simulink model "non_ACC"  (R2021b)
settings: Solver=ode5  StartTime=0.0  StopTime=90  FixedStep=1/20  RelTol=1e-3
PreLoadFcn:
  | mbxruntime.callbacks.PreLoadFcn(bdroot);
PostLoadFcn:
  | mbxruntime.callbacks.PostLoadFcn(bdroot);
InitFcn:
  | mbxruntime.callbacks.InitFcn(bdroot);
StartFcn:
  | mbxruntime.callbacks.StartFcn(bdroot);
StopFcn:
  | mbxruntime.callbacks.StopFcn(bdroot);
model workspace: external: MAT-File .\kea_demo_0218_cs_hws.mat (data not in the file)
undefined symbols (not defined in the file): DiscIntNeverNeededParam, kea_demo_0218_cs_1d5c9b61e8e009e5, kea_demo_0218_cs_4669f259e7287783, kea_demo_0218_cs_87ee11d7829c0052, kea_demo_0218_cs_Audi_A3_1_Dynamics_Simple_initialPitch, kea_demo_0218_cs_Audi_A3_1_Dynamics_Simple_initialRoll, kea_demo_0218_cs_Audi_A3_1_Dynamics_Simple_initialX, kea_demo_0218_cs_Audi_A3_1_Dynamics_Simple_initialY, kea_demo_0218_cs_Audi_A3_1_Dynamics_Simple_initialYaw, kea_demo_0218_cs_Audi_A3_1_Dynamics_Simple_initialZ, kea_demo_0218_cs_Audi_A3_1_PathFollower_Preview_1_PathUniqueID, kea_demo_0218_cs_Roewe_550_S_Sedan_1_Dynamics_Simple_initialX, kea_demo_0218_cs_Roewe_550_S_Sedan_1_Dynamics_Simple_initialY, kea_demo_0218_cs_Roewe_550_S_Sedan_1_Dynamics_Simple_initialYaw, kea_demo_0218_cs_Roewe_550_S_Sedan_1_Dynamics_Simple_initialZ, mbxruntime, warningInitialVelocity, x0
libraries: simulink x56, simulink_extras x18
(part 1 of 7)
CloseFcn:
  | mbxruntime.callbacks.CloseFcn(bdroot);
settings Model: PacingRate=10  Creator=PRESCAN  LastModifiedBy=PRO
settings SolverCC: AlgebraicLoopSolver=TrustRegion
settings DataIOCC: LimitDataPoints=on  SaveFormat=Array  SignalLoggingSaveFormat=ModelDataLogs  ReturnWorkspaceOutputs=off
settings OptimizationCC: DefaultParameterBehavior=Inlined  ExpressionDepthLimit=2147483647  InitFltsAndDblsToZero=on  LifeSpan=inf
settings DebuggingCC: SaveWithParameterizedLinksMsg=none  UnderspecifiedInitializationDetection=Classic  MergeDetectMultiDrivingBlocksExec=none  SignalResolutionControl=TryResolveAllWithWarning  MultiTaskDSMMsg=warning  MultiTaskCondExecSysMsg=none  FcnCallInpInsideContextMsg=warning  AllowSymbolicDim=off  StateNameClashWarn=warning  SFUnexpectedBacktrackingDiag=warning  SFNoUnconditionalDefaultTransitionDiag=warning  SFExecutionAtInitializationDiag=none  SFMachineParentedDataDiag=warning  ArithmeticOperatorsInVariantConditions=warning
settings HardwareCC: ProdBitPerPointer=32  ProdBitPerSizeT=32  ProdBitPerPtrDiffT=32  ProdLargestAtomicFloat=None  ProdIntDivRoundTo=Undefined  ProdEndianess=Unspecified  ProdWordSize=32  ProdHWDeviceType=32-bit Generic
settings ModelReferenceCC: UpdateModelReferenceTargets=IfOutOfDate  PropagateSignalLabelsOutOfModel=off
settings SFSimCC: SimUseLocalCustomCode=off  SimParseCustomCode=off  CustomCodeUndefinedFunction=UseInterfaceOnly
settings SFSimCC: SimCustomHeaderCode=|
  | #include "prescan.h"
  | #include "prescan_platform.h"
settings RTWCC: RTWUseLocalCustomCode=off
settings CodeAppCC: StateflowObjectComments=on
settings GRTTargetCC: TargetFcnLib=ansi_tfl_tmw.mat  TargetLangStandard=C89/C90 (ANSI)  CombineOutputUpdateFcns=off  GRTInterface=on
settings ConfigComp: CovMetricSettings=dw  CovSaveCumulativeToWorkspaceVar=on  CovSaveSingleToWorkspaceVar=on  CovExternalEMLEnable=off  CovSFcnEnable=off

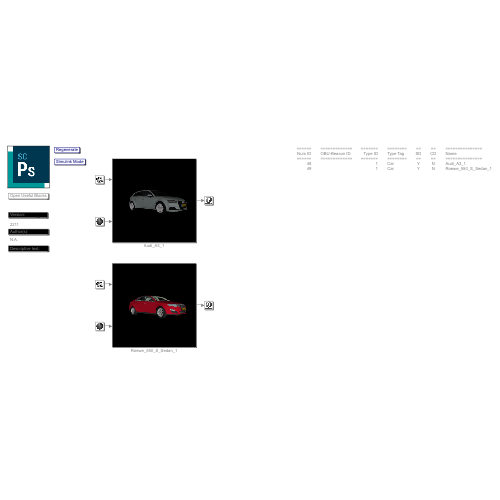
[thumbnail: Simulink's stored preview of the top-level diagram]
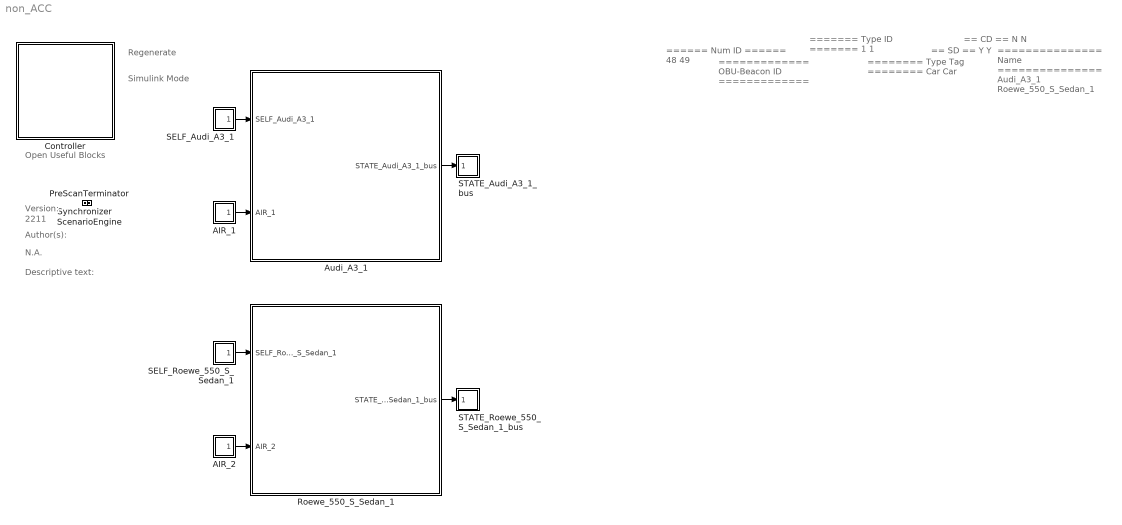
== system non_ACC ==
  note: Regenerate
  note: Simulink Mode
  note: Open Useful Blocks
  note: 2211
  note: Version:
  note: Author(s):
  note: N.A.
  note: Descriptive text:
  note: ======
      | Num ID
      | ======
      | 48
      | 49
  note: =============
      | OBU-Beacon ID
      | =============
  note: =======
      | Type ID
      | =======
      | 1
      | 1
  note: ========
      | Type Tag
      | ========
      | Car
      | Car
  note: ==
      | SD
      | ==
      | Y
      | Y
  note: ==
      | CD
      | ==
      | N
      | N
  note: ===============
      | Name
      | ===============
      | Audi_A3_1
      | Roewe_550_S_Sedan_1
  AIR_1 : Subsystem  Tag=sensor/AIR  Priority=30  LoadFcn=load('PrescanAIRSensorData.mat');load('PrescanAIRSensorMessage.mat')  mask(PreScan Source Block: Actor Independent Receiver (AIR)){}
      mask help:
      | The Actor Information Receiver sensor provides a fast, simple and generic detection solution which is not tied up to a specific technology. The AIR detects the intersection point of the bounding box with the straight line from the sensor axis system to the middle of the bounding box.
      |
      | For more information, please click Help.
      settings: OpenFcn=open_system([gcb '/Sensor'],'mask')
      mask Help: eval('openHelp(413)')
      mask Display: image(imread('AIR.png'))
  AIR_2 : Subsystem  Tag=sensor/AIR  Priority=30  LoadFcn=load('PrescanAIRSensorData.mat');load('PrescanAIRSensorMessage.mat')  mask(PreScan Source Block: Actor Independent Receiver (AIR)){}
      mask help:
      | The Actor Information Receiver sensor provides a fast, simple and generic detection solution which is not tied up to a specific technology. The AIR detects the intersection point of the bounding box with the straight line from the sensor axis system to the middle of the bounding box.
      |
      | For more information, please click Help.
      settings: OpenFcn=open_system([gcb '/Sensor'],'mask')
      mask Help: eval('openHelp(413)')
      mask Display: image(imread('AIR.png'))
  Audi_A3_1 : Subsystem  Tag=WorldObjectSubSystem  InitFcn=UniqueId = '189';
      mask init:
      | modelPath = GenericModelHelper.getGenericModelFilePath('ModelDepo','Vehicles\Audi_A3\Audi_A3.pgmb','904257d8a4712c49871b2bb1a5c4c7b1');imagePath = GenericModelHelper.getCompilationPicture(modelPath, 'Audi_A3.png');
      mask Display: image(imread(imagePath));color('white');text(0, 0, ' ID=48\n')
  Controller : Subsystem  Description=8A3CD2955739A82C886C20AE3E253D78460D53180EE2C1B14CC08DF75A70BE77  Priority=-1  LoadFcn=load PreScanControllerData  mask(PreScan Simulation Controller){prescanversion='2022.3.0', ModelReferencing=off, TimeStep=1/20, ControlMode=0, PreScanExecutionMode=on, ControllerCount=0, ControllerIndex=0, ControllerOptions=''}
      mask prompts: prescanversion "Prescan Version"; ModelReferencing "Use Model Referencing"; TimeStep "Upload Period [s]"; ControlMode "Control Mode"; PreScanExecutionMode "Execution Mode"; ControllerCount "Controller Count"; ControllerIndex "Controller Index"; ControllerOptions "Controller Options"
      mask help:
      | Please do not remove this block from the compilation sheet,
      | as it connects the model to the Prescan environment.
      mask init:
      | model = bdroot(gcb);
      | ExperimentFile = mbxruntime.findExperimentFile(model,true); %relative path
      | 
      | [d1, d2, prescandata] = prescan_Settings();
      | ModelDepo = fullfile(prescandata,'ModelDepo'); 
      | 
      | RTmode = mbxruntime.getRTMode(model);
      | 
      | SimulationMode = get_param(bdroot,'SimulationMode');
      | if strcmp(SimulationMode, 'rapid-accelerator')
      |     SimulationMode = 'external';
      | end
      | TargetName = get_param(bdroot,'SystemTargetFile');
      settings: ModelCloseFcn=assignin('base',['model_closed_' bdroot],true);
      mask Help: eval('openHelp(812)')
      mask Display: image(imread('prescanlogo.ico'))
  PreScanTerminator : Subsystem  Tag=PreScanTerminator  Priority=999  LoadFcn=load PrescanTerminatorData  mask(PreScan Simulation Terminator){TimeStep=1/20}
      mask prompts: TimeStep "Upload Period [s]"
      mask help:
      | Please do not remove this block from the compilation sheet as it
      | connects the model to the PreScan environment.
      mask Help: eval('openHelp(812)')
      mask Display: image(imread('prescanlogo.ico'))
  Roewe_550_S_Sedan_1 : Subsystem  Tag=WorldObjectSubSystem  InitFcn=UniqueId = '192';
      mask init:
      | modelPath = GenericModelHelper.getGenericModelFilePath('ModelDepo','Vehicles\Roewe_550_S\Roewe_550_S.pgmb','e36b3c1cdc77adba028a993f0879aa02');imagePath = GenericModelHelper.getCompilationPicture(modelPath, 'Roewe_550_S_HighPoly.png');
      mask Display: image(imread(imagePath));color('white');text(0, 0, ' ID=49\n')
  SELF_Audi_A3_1 : Subsystem  Tag=sensor/SelfPort  Priority=30  LoadFcn=load('PreScanSelfSensorData.mat')  mask(PreScan Source Block: SELF){}
      mask help:
      | The SELF port shows (state) information of the actor itself. The outputs are position in the experiment's axis system and the GPS coordinates, and the object's absolute velocity and compass heading.
      |
      | For more information, please click Help.
      settings: OpenFcn=open_system([gcb '/Sensor'],'mask')
      mask Help: eval('openHelp(462)')
      mask Display: image(imread('GPS.png'))
  SELF_Roewe_550_S_Sedan_1 : Subsystem  Tag=sensor/SelfPort  Priority=30  LoadFcn=load('PreScanSelfSensorData.mat')  mask(PreScan Source Block: SELF){}
      mask help:
      | The SELF port shows (state) information of the actor itself. The outputs are position in the experiment's axis system and the GPS coordinates, and the object's absolute velocity and compass heading.
      |
      | For more information, please click Help.
      settings: OpenFcn=open_system([gcb '/Sensor'],'mask')
      mask Help: eval('openHelp(462)')
      mask Display: image(imread('GPS.png'))
  STATE_Audi_A3_1_bus : Subsystem  Tag=actuator/StatePort  Priority=0  LoadFcn=load('PreScanStateActuatorData.mat')  mask(PreScan Sink Block: State){}
      mask help:
      | The Actor State contains a vector signal of size (9x1), containing the following signals:
      |
      | -  Position    	(x,y,z)             	[m]
      | -  Velocity    	(vx,vy,vz)         	[m/s]
      | -  Angles       	(Roll, Pitch, Yaw)	[rad]
      |
      | The Actor state is defined in the global axis system.
      | The state is superponed on the Initial position defined in the GUI.
      |
      | For more information, please click Help.
      settings: OpenFcn=open_system([gcb '/Actuator'],'mask')
      mask Help: eval('openHelp(222)')
      mask Display: image(imread('State.png'))
  STATE_Roewe_550_S_Sedan_1_bus : Subsystem  Tag=actuator/StatePort  Priority=0  LoadFcn=load('PreScanStateActuatorData.mat')  mask(PreScan Sink Block: State){}
      mask help:
      | The Actor State contains a vector signal of size (9x1), containing the following signals:
      |
      | -  Position    	(x,y,z)             	[m]
      | -  Velocity    	(vx,vy,vz)         	[m/s]
      | -  Angles       	(Roll, Pitch, Yaw)	[rad]
      |
      | The Actor state is defined in the global axis system.
      | The state is superponed on the Initial position defined in the GUI.
      |
      | For more information, please click Help.
      settings: OpenFcn=open_system([gcb '/Actuator'],'mask')
      mask Help: eval('openHelp(222)')
      mask Display: image(imread('State.png'))
  ScenarioEngine : Subsystem  Tag=PreScanOpenScenarioBlock  Priority=10  LoadFcn=load PrescanSynchronizeData  mask(PreScan Simulation Core Block){TimeStep=1/20}
      mask prompts: TimeStep "Timestep [s]"
      mask help:
      | Please do not remove this block from the PreScan compilation sheet,
      | as it contains essential configuration parameters for a PreScan simulation.
      settings: DeleteFcn=PreScanBlockDeleteFcn;
      mask Display: image(imread('prescanlogo.ico'))
  Synchronizer : Subsystem  Tag=PreScanSynchronizer  Priority=20  LoadFcn=load PrescanSynchronizeData  mask(PreScan Simulation Core Block){TimeStep=1/20}
      mask prompts: TimeStep "Timestep [s]"
      mask help:
      | Please do not remove this block from the PreScan compilation sheet,
      | as it contains essential configuration parameters for a PreScan simulation.
      settings: DeleteFcn=PreScanBlockDeleteFcn;
      mask Display: image(imread('prescanlogo.ico'))
  wires:
  Audi_A3_1/1(STATE_Audi_A3_1_bus) -> STATE_Audi_A3_1_bus/1(STATE_Audi_A3_1_bus)
  SELF_Audi_A3_1/1(SELF_Audi_A3_1) -> Audi_A3_1/1(SELF_Audi_A3_1)
  AIR_1/1(AIR_1) -> Audi_A3_1/2(AIR_1)
  Roewe_550_S_Sedan_1/1(STATE_Roewe_550_S_Sedan_1_bus) -> STATE_Roewe_550_S_Sedan_1_bus/1(STATE_Roewe_550_S_Sedan_1_bus)
  SELF_Roewe_550_S_Sedan_1/1(SELF_Roewe_550_S_Sedan_1) -> Roewe_550_S_Sedan_1/1(SELF_Roewe_550_S_Sedan_1)
  AIR_2/1(AIR_2) -> Roewe_550_S_Sedan_1/2(AIR_2)

== system non_ACC/AIR_1 ==
  Sensor : S-Function  FunctionName=sfun_AIRSensor  Parameters=mbxruntime.parameters.convert(detectableObjects), mbxruntime.parameters.convert(sensorID), mbxruntime.parameters.convert(timestep)  SFunctionDeploymentMode=off  EnableBusSupport=off  mask(PreScan Source Block: Actor Independent Receiver (AIR)){detectableObjects=1, sensorID=190, timestep=1/20}
      mask prompts: detectableObjects "Max detectable objects"; sensorID "Sensor ID"; timestep "MATLAB timestep:"
      mask help:
      | The Actor Information Receiver sensor provides a fast, simple and generic detection solution which is not tied up to a specific technology. The AIR detects the intersection point of the bounding box with the straight line from the sensor axis system to the middle of the bounding box.
      |
      | For more information, please click Help.
      mask Help: eval('openHelp(413)')
      mask Display: image(imread('AIR.png'))
  AIR_1 : Outport  Tag=outport/AIR  OutDataTypeStr=Bus: PRESCAN_AIRSENSORMESSAGE  PortDimensions=1  SampleTime=1/20
  wires:
  Sensor/1 -> AIR_1/1

== system non_ACC/AIR_2 ==
  Sensor : S-Function  FunctionName=sfun_AIRSensor  Parameters=mbxruntime.parameters.convert(detectableObjects), mbxruntime.parameters.convert(sensorID), mbxruntime.parameters.convert(timestep)  SFunctionDeploymentMode=off  EnableBusSupport=off  mask(PreScan Source Block: Actor Independent Receiver (AIR)){detectableObjects=1, sensorID=193, timestep=1/20}
      mask prompts: detectableObjects "Max detectable objects"; sensorID "Sensor ID"; timestep "MATLAB timestep:"
      mask help:
      | The Actor Information Receiver sensor provides a fast, simple and generic detection solution which is not tied up to a specific technology. The AIR detects the intersection point of the bounding box with the straight line from the sensor axis system to the middle of the bounding box.
      |
      | For more information, please click Help.
      mask Help: eval('openHelp(413)')
      mask Display: image(imread('AIR.png'))
  AIR_2 : Outport  Tag=outport/AIR  OutDataTypeStr=Bus: PRESCAN_AIRSENSORMESSAGE  PortDimensions=1  SampleTime=1/20
  wires:
  Sensor/1 -> AIR_2/1

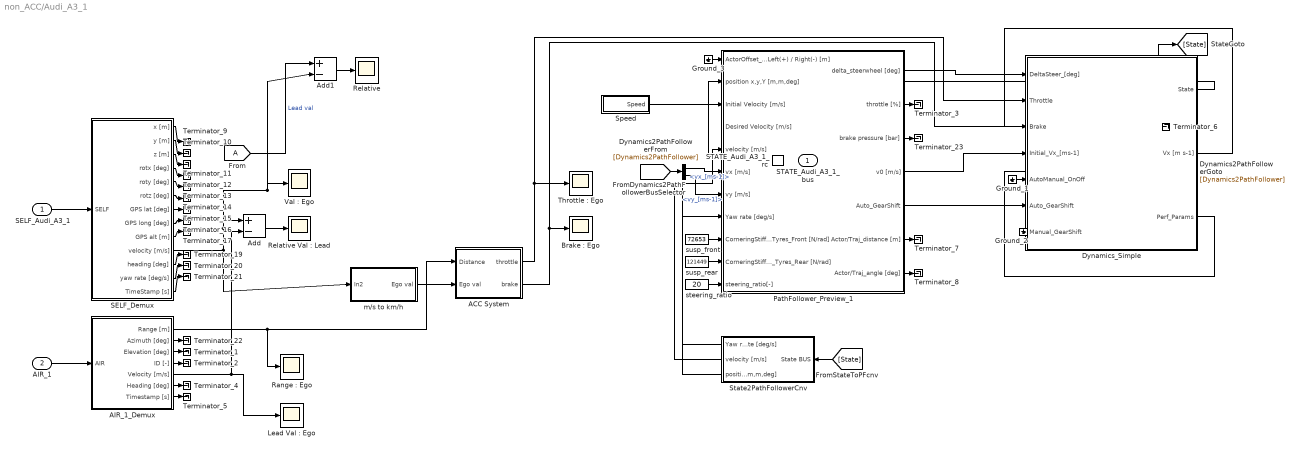
== system non_ACC/Audi_A3_1 ==
  SELF_Audi_A3_1 : Inport  Tag=inport/SelfPort  OutDataTypeStr=Bus: PRESCAN_SELFSENSORDATA  PortDimensions=1  SampleTime=1/20  BusOutputAsStruct=on
  AIR_1 : Inport  Tag=inport/AIR  Port=2  OutDataTypeStr=Bus: PRESCAN_AIRSENSORMESSAGE  PortDimensions=1  SampleTime=1/20  BusOutputAsStruct=on
  ACC System : Subsystem
  AIR_1_Demux : Subsystem  Tag=demux/AIR  mask(PreScan Demux Block: AIR){DetectionType=BBox, detectableObjects=1}
      mask prompts: DetectionType "Detection Type"; detectableObjects "Max. detectable objects"
      mask help:
      | The Actor Information Receiver sensor provides a fast, simple and generic detection solution which is not tied up to a specific technology and can be used for scenarios in which a simple sensor is needed.
      |
      | For more information, please click Help.
      mask init:
      | switch DetectionType
      |     case 1
      |         DetectionTypeStr = 'Center';
      |     case 2
      |         DetectionTypeStr = 'BBox';
      |     case 3
      |         DetectionTypeStr = 'CoG';
      |     otherwise
      |         DetectionTypeStr = 'Unknown';
      | end
      settings: DeleteFcn=PreScanBlockDeleteFcn;
      mask Help: eval('openHelp(413)')
      mask TypeOptions DetectionType: Center | BBox | CoG
      mask Display:
      | disp(char('Det. type:         ',['{\it',DetectionTypeStr,'}']),'texmode','on')
      | port_label('output',1,'Range [m]')
      | port_label('output',2,'{\theta} [deg]','texmode','on')
      | port_label('output',3,'{\phi} [deg]','texmode','on')
      | port_label('output',4,'ID [-]','texmode','on')
      | port_label('output',5,'Velocity [m/s]','texmode','on')
      | port_label('output',6,'Heading [deg]','texmode','on')
      | port_label('output',7,'Timestamp [s]','texmode','on')
  Add : Sum  Inputs=+-
  Add1 : Sum  Inputs=+-
  "Brake : Ego" : Scope
  Dynamics_Simple : Subsystem  Tag=Simple_Vehicle_Dynamics  mask(PreScan Block: Simple Dynamics){TimeStep=1/20, initialX=kea_demo_0218_cs_Audi_A3_1_Dynamics_Simple_initialX, initialY=kea_demo_0218_cs_Audi_A3_1_Dynamics_Simple_initialY, initialZ=kea_demo_0218_cs_Audi_A3_1_Dynamics_Simple_initialZ, initialRoll=kea_demo_0218_cs_Audi_A3_1_Dynamics_Simple_initialRoll, initialPitch=kea_demo_0218_cs_Audi_A3_1_Dynamics_Simple_initialPitch, initialYaw=kea_demo_0218_cs_Audi_A3_1_Dynamics_Simple_initialYaw}
      mask prompts: TimeStep "Auto assigned: Time Step [s]"; initialX "Ini x-position VEHICLE wrt GLOBAL axis system [m]"; initialY "Ini y-position VEHICLE wrt GLOBAL axis system [m]"; initialZ "Ini z-position VEHICLE wrt GLOBAL axis system [m]"; initialRoll "Ini roll-angle BODY wrt VEHICLE axis system [deg]"; initialPitch "Ini pitch-angle BODY wrt VEHICLE axis system [deg]"; initialYaw "Ini yaw-angle VEHICLE wrt GLOBAL axis system [deg]"
      mask help:
      | The Simple Dynamics Model is selected in the GUI to simulate vehicle dynamics behavior.
      |
      | The Simple Dynamics Model is completely open to the user. The parameters of this model can be set in the Simple Dynamics dialog in the GUI.
      |
      | For more information, please click Help.
      mask init:
      | p = SimpleDyn_pars;
      settings: DeleteFcn=PreScanBlockDeleteFcn;
      mask Help: eval('openHelp(220)')
      mask Display:
      | image(imread('SimpleDyn.png'))
      | port_label('input', 1, '{\delta}_S_t_ _e_e_r [deg]','texmode','on')
      | port_label('input', 2, 'Throttle [%]')
      | port_label('input', 3, 'Brake Pres [bar]')
      | port_label('input', 4, 'V_0 [ms-1]','texmode','on')
      | port_label('input', 5, 'Auto=[0]/Manual=[1]')
      | port_label('input', 6, 'Auto_GearShift')
      | port_label('input', 7, 'Manual_GearShift')
      | port_label('output', 1, 'State')
      | port_label('output', 2, 'Vx [ms-1]')
      | port_label('output', 3, 'Perf Params')
  FromDynamics2PathFollowerBusSelector : BusSelector  OutputSignals=vx_[ms-1],vy_[ms-1]
  Ground_1 : Ground
  Ground_2 : Ground
  Ground_3 : Ground
  "Lead Val : Ego" : Scope
  PathFollower_Preview_1 : Subsystem  Tag=PathFollower_Preview  LoadFcn=load PrescanXYZData;  mask(PreScan Block: Path Follower with Preview){LongCtrl_P=20, LongCtrl_I=0.3, LongCtrl_D=3.065, LongCtrl_AWU=1, LongCtrlDefault_P=20, LongCtrlDefault_I=0.3, LongCtrlDefault_D=3.065, LongCtrlDefault_AWU=1, PathUniqueID=kea_demo_0218_cs_Audi_A3_1_PathFollower_Preview_1_PathUniqueID, mass=1820, Jzz=3746, length_a=1.34, length_l=2.609, Angle_Max_SteeringWheel=500, PreviewTime=1, DelayTime=0.1, LowSpeedLimit=20, MaxSteeringRate=1200, CSSampleTime=1/20, PFIntegrationFrequency=20}
      mask prompts: LongCtrl_P "Longitudinal Controller P"; LongCtrl_I "Longitudinal Controller I"; LongCtrl_D "Longitudinal Controller D"; LongCtrl_AWU "Longitudinal Controller AWU"; PathUniqueID "Path Unique ID"; mass "Mass vehicle total [kg]"; Jzz "Inertia vehicle around yaw axis [kg m2]"; length_a "Distance between COG and front axle [m]"; length_l "Length of wheelbase [m]"; Angle_Max_SteeringWheel "Maximum steering wheel angle [deg]"; PreviewTime "Preview time [s]"; DelayTime "Delay time [s]"; LowSpeedLimit "Low-speed limit [km/h]"; MaxSteeringRate "Maximum steering wheel angle rate [deg/s]"; CSSampleTime "Compilation Sheet sample time [s]"; PFIntegrationFrequency "Lateral controller frequency [Hz]"
      mask help:
      | The Path Follower Model is selected in the GUI to simulate driver behavior.
      |
      | For more information, please click Help.
      mask init:
      | RefreshCounter = max(floor((1/CSSampleTime) / (PFIntegrationFrequency)), 1);
      | PathFollowerBlockPath = gcb;
      mask Help: eval('openHelp(233)')
      mask DialogControl Container12 Prompt: Controller Parameters
      mask DialogControl Control2 Prompt: Reset PID parameters
      mask DialogControl Control2 Callback:
      | LongCtrlDefault_P = get_param(gcb,'LongCtrlDefault_P');
      | set_param(gcb,'LongCtrl_P',LongCtrlDefault_P);
      | 
      | LongCtrlDefault_I = get_param(gcb,'LongCtrlDefault_I');
      | set_param(gcb,'LongCtrl_I',LongCtrlDefault_I);
      | 
      | LongCtrlDefault_D = get_param(gcb,'LongCtrlDefault_D');
      | set_param(gcb,'LongCtrl_D',LongCtrlDefault_D);
      | 
      | LongCtrlDefault_AWU = get_param(gcb,'LongCtrlDefault_AWU');
      | set_param(gcb,'LongCtrl_AWU',LongCtrlDefault_AWU);
      mask DialogControl Container10 Prompt: System Parameters
  "Range : Ego" : Scope
  Relative : Scope
  "Relative Val : Lead" : Scope
  SELF_Demux : Subsystem  Tag=demux/SelfPort  mask(PreScan Demux Block:){}
      mask help:
      | The SELF port shows (state) information of the actor itself. The outputs are position in the experiment's axis system and the GPS coordinates, and the object's absolute velocity and compass heading.
      |
      | For more information, please click Help.
      settings: DeleteFcn=PreScanBlockDeleteFcn;
      mask Help: eval('openHelp(462)')
      mask Display:
      | port_label('output',1,'x [m]')
      | port_label('output',2,'y [m]')
      | port_label('output',3,'z [m]','texmode','on')
      | port_label('output',4,'Rotx [deg]','texmode','on')
      | port_label('output',5,'Roty [deg]','texmode','on')
      | port_label('output',6,'Rotz [deg]','texmode','on')
      | port_label('output',7,'GPS lat [deg]','texmode','on')
      | port_label('output',8,'GPS long [deg]','texmode','on')
      | port_label('output',9,'GPS alt [m]','texmode','on')
      | port_label('output',10,'Velocity [m/s]')
      | port_label('output',11,'Heading [deg]')
      | port_label('output',12,'Yaw rate [deg/s]')
      | port_label('output',13,'Timestamp [s]')
  STATE_Audi_A3_1_rc : RateTransition  Tag=mux_rc/StatePort  OutPortSampleTimeOpt=Inherit
  Speed : Subsystem
      settings: OpenFcn=open_system([gcb '/sfun'],'mask')
  State2PathFollowerCnv : Subsystem  Tag=State2PFConnection/cnv
  Terminator_{1..17,19..23} (22 alike) : Terminator
  "Throttle : Ego" : Scope
  "Val : Ego" : Scope
  m/s to km/h : Subsystem
  steering_ratio : Constant  Tag=steering_ratio  Value=20
  susp_front : Constant  Tag=susp_front  Value=72653
  susp_rear : Constant  Tag=susp_rear  Value=121449
  STATE_Audi_A3_1_bus : Outport  Tag=outport/StatePort  OutDataTypeStr=Bus: PRESCAN_STATEACTUATORDATA  PortDimensions=1  SampleTime=1/20
  wires:
  STATE_Audi_A3_1_rc/1 -> STATE_Audi_A3_1_bus/1
  SELF_Audi_A3_1/1 -> SELF_Demux/1(SELF)
  AIR_1/1 -> AIR_1_Demux/1(AIR)
  susp_front/1 -> PathFollower_Preview_1/9(CorneringStiffness_Tyres_Front [N/rad])
  susp_rear/1 -> PathFollower_Preview_1/10(CorneringStiffness_Tyres_Rear [N/rad])
  steering_ratio/1 -> PathFollower_Preview_1/11(steering_ratio[-])
  Speed/1(Speed) -> PathFollower_Preview_1/3(Initial Velocity [m/s])
  Dynamics_Simple/1(State) -> STATE_Audi_A3_1_rc/1, [State]
  [State] -> State2PathFollowerCnv/1(State BUS)
  State2PathFollowerCnv/1(Yaw rate [deg/s]) -> PathFollower_Preview_1/8(Yaw rate [deg/s])
  State2PathFollowerCnv/2(velocity [m/s]) -> PathFollower_Preview_1/5(velocity [m/s])
  State2PathFollowerCnv/3(position x,y,Y [m,m,deg]) -> PathFollower_Preview_1/2(position x,y,Y [m,m,deg])
  PathFollower_Preview_1/1(delta_steerwheel [deg]) -> Dynamics_Simple/1(DeltaSteer_[deg])
  PathFollower_Preview_1/2(throttle [%]) -> Terminator_3/1
  PathFollower_Preview_1/3(brake pressure [bar]) -> Terminator_23/1
  PathFollower_Preview_1/4(v0 [m/s]) -> Dynamics_Simple/4(Initial_Vx_[ms-1])
  PathFollower_Preview_1/5(Auto_GearShift) -> Dynamics_Simple/6(Auto_GearShift)
  Dynamics_Simple/3(Perf_Params) -> [Dynamics2PathFollower]
  FromDynamics2PathFollowerBusSelector/1 -> PathFollower_Preview_1/6(vx [m/s])  "<vx_[ms-1]>"
  FromDynamics2PathFollowerBusSelector/2 -> PathFollower_Preview_1/7(vy [m/s])  "<vy_[ms-1]>"
  [Dynamics2PathFollower] -> FromDynamics2PathFollowerBusSelector/1
  AIR_1_Demux/3(Elevation [deg]) -> Terminator_1/1
  AIR_1_Demux/4(ID [-]) -> Terminator_2/1
  AIR_1_Demux/6(Heading [deg]) -> Terminator_4/1
  AIR_1_Demux/7(Timestamp [s]) -> Terminator_5/1
  Ground_1/1 -> Dynamics_Simple/5(AutoManual_OnOff)
  Ground_2/1 -> Dynamics_Simple/7(Manual_GearShift)
  Dynamics_Simple/2(Vx [m s-1]) -> Terminator_6/1
  Ground_3/1 -> PathFollower_Preview_1/1(ActorOffset_Left(+) / Right(-) [m])
  PathFollower_Preview_1/6(Actor/Traj_distance [m]) -> Terminator_7/1
  PathFollower_Preview_1/7(Actor/Traj_angle [deg]) -> Terminator_8/1
  SELF_Demux/1(x [m]) -> Terminator_9/1
  SELF_Demux/2(y [m]) -> Terminator_10/1
  SELF_Demux/3(z [m]) -> Terminator_11/1
  SELF_Demux/4(rotx [deg]) -> Terminator_12/1
  SELF_Demux/5(roty [deg]) -> Terminator_13/1
  SELF_Demux/6(rotz [deg]) -> Terminator_14/1
  SELF_Demux/7(GPS lat [deg]) -> Terminator_15/1
  SELF_Demux/8(GPS long [deg]) -> Terminator_16/1
  SELF_Demux/9(GPS alt [m]) -> Terminator_17/1
  SELF_Demux/11(heading [deg]) -> Terminator_19/1
  SELF_Demux/12(yaw rate [deg/s]) -> Terminator_20/1
  SELF_Demux/13(TimeStamp [s]) -> Terminator_21/1
  AIR_1_Demux/2(Azimuth [deg]) -> Terminator_22/1
  AIR_1_Demux/1(Range [m]) -> "Range : Ego"/1, ACC System/1(Distance)
  ACC System/1(throttle) -> Dynamics_Simple/2(Throttle), "Throttle : Ego"/1
  ACC System/2(brake) -> Dynamics_Simple/3(Brake), "Brake : Ego"/1
  m/s to km/h/1(Ego val) -> ACC System/2(Ego val)
  Add/1 -> "Relative Val : Lead"/1
  SELF_Demux/10(velocity [m/s]) -> Add/1, Add1/2, "Val : Ego"/1, m/s to km/h/1(In2)
  AIR_1_Demux/5(Velocity [m/s]) -> "Lead Val : Ego"/1, Add/2
  Add1/1 -> Relative/1
  [A] -> Add1/1  "Lead val"

== system non_ACC/Controller ==
  Terminator : Terminator
  sfun_Controller : S-Function  FunctionName=sfun_Controller  Parameters=SParameter1, SParameter2, SParameter3, SParameter4, SParameter5, SParameter6, SParameter7, SParameter8, SParameter9, SParameter10, SampleTime  SFunctionDeploymentMode=off  EnableBusSupport=off  mask(Legacy Function){SFunctionSpec=void prescan_outputFcn(void** work1, PRESCAN_CONTROLLERDATA y1[1]), SParameter1=uint8([ExperimentFile 0]), SParameter2=uint8([ModelDepo 0]), SParameter3=uint8([ControllerOptions 0]), SParameter4=RTmode, SParameter5=PreScanExecutionMode, SParameter6=ControlMode, SParameter7=ControllerCount, SParameter8=ControllerIndex, SParameter9=uint8([SimulationMode 0]), SParameter10=uint8([TargetName 0]), SampleTime=TimeStep, ShowSpec=on}
      mask prompts: SParameter1 "P1:"; SParameter2 "P2:"; SParameter3 "P3:"; SParameter4 "P4:"; SParameter5 "P5:"; SParameter6 "P6:"; SParameter7 "P7:"; SParameter8 "P8:"; SParameter9 "P9:"; SParameter10 "P10:"; SampleTime "Sample time (-1 for inherited):"; ShowSpec "Display function specification"
      mask help:
      | This block allows you to call the legacy functions specified by the following Legacy Code Tool definition:
      | def.SFunctionName = 'sfun_Controller';
      | def.OutputFcnSpec = 'void prescan_outputFcn(void** work1, PRESCAN_CONTROLLERDATA y1[1])';
      | def.StartFcnSpec = 'void prescan_startFcn(void ** work1, uint8 p1[], uint8 p2[], uint8 p3[], double p4, double p5, double p6, double p7, double p8, uint8 p9[], uint8 p10[])';
      | def.TerminateFcnSpec = 'void prescan_terminateFcn(void** work1)';
      | def.HeaderFiles = {'prescan_controller_data.h', 'prescan_SFunLibrary.h', 'prescan_CreateLogHandler.h', 'prescan_CreateErrorHandler.h', 'prescan_modify.h', 'ModuleDLL.h'};
      | def.SourceFiles = {'prescan_MexLogHandler.c', 'prescan_SimStructErrorHandler.c', 'prescan_ErrorHandler.c', 'prescan_Modify.c'};
      | def.HostLibFiles = {'sensorinterfaced.lib'};
      | def.TargetLibFiles = {'sensorinterfaced.so'};
      | def.IncPaths = {'.', 'C:\projects\prescan\rt_vislibrary\vis\..\pimp\include\sensors\InterfaceRTW'};
      | def.SrcPaths = {'C:\projects\prescan\rt_vislibrary\vis\..\pimp\include\sensors\InterfaceRTW', 'C:\projects\prescan\rt_vislibrary\vis\..\pimp\include\sensors\InterfaceRTW\ccurrt'};
      | def.LibPaths = {'C:\\projects\\prescan\\vislibrary_build\lib'};
      | def.SampleTime = 'parameterized';
      mask Help: <p>This block was generated automatically by the Legacy Code Tool. For detailed help on this tool, call<a href="matlab:legacy_code('help')"> legacy_code('help')</a>.</p>
      mask Callback ShowSpec:
      | if strcmp(get_param(gcbh, 'ShowSpec'), 'on')
      |   set_param(gcbh, 'MaskDisplay', sprintf('fprintf(''%s'');', get_param(gcbh, 'SFunctionSpec')));
      | else
      |   set_param(gcbh, 'MaskDisplay', sprintf('fprintf(''%s'');', get_param(gcbh, 'FunctionName')));
      | end
      mask Display: fprintf('void prescan_outputFcn(void** work1, PRESCAN_CONTROLLERDATA y1[1])');
  wires:
  sfun_Controller/1 -> Terminator/1

== system non_ACC/PreScanTerminator ==
  Terminator : Terminator
  sfun_Terminator : S-Function  FunctionName=sfun_Terminator  Parameters=SampleTime  SFunctionDeploymentMode=off  EnableBusSupport=off  mask(Legacy Function){SFunctionSpec=void prescan_terminator_outputFcn(void ** work1, PRESCAN_TERMINATORDATA y1[1]), SampleTime=TimeStep, ShowSpec=on}
      mask prompts: SampleTime "Sample time (-1 for inherited):"; ShowSpec "Display function specification"
      mask help:
      | This block allows you to call the legacy functions specified by the following Legacy Code Tool definition:
      | def.SFunctionName = 'sfun_Terminator';
      | def.OutputFcnSpec = 'void prescan_terminator_outputFcn(void ** work1, PRESCAN_TERMINATORDATA y1[1])';
      | def.StartFcnSpec = 'void prescan_terminator_startFcn(void ** work1)';
      | def.TerminateFcnSpec = 'void prescan_terminator_terminateFcn(void ** work1)';
      | def.HeaderFiles = {'prescan_terminator_data.h'};
      | def.HostLibFiles = {'sensorinterfaced.lib'};
      | def.IncPaths = {'src', 'C:\prescandev\vislibrary\vis\..\pimp\include\sensors\InterfaceRTW'};
      | def.SrcPaths = {'src'};
      | def.LibPaths = {'C:\\prescandev\\vislibrary_build\lib'};
      | def.SampleTime = 'parameterized';
      | def.Options.language = 'C';
      mask Help: <p>This block was generated automatically by the Legacy Code Tool. For detailed help on this tool, call<a href="matlab:legacy_code('help')"> legacy_code('help')</a>.</p>
      mask Callback ShowSpec:
      | if strcmp(get_param(gcbh, 'ShowSpec'), 'on')
      |   set_param(gcbh, 'MaskDisplay', sprintf('fprintf(''%s'');', get_param(gcbh, 'SFunctionSpec')));
      | else
      |   set_param(gcbh, 'MaskDisplay', sprintf('fprintf(''%s'');', get_param(gcbh, 'FunctionName')));
      | end
      mask Display: fprintf('void prescan_terminator_outputFcn(void ** work1, PRESCAN_TERMINATORDATA y1[1])');
  wires:
  sfun_Terminator/1 -> Terminator/1

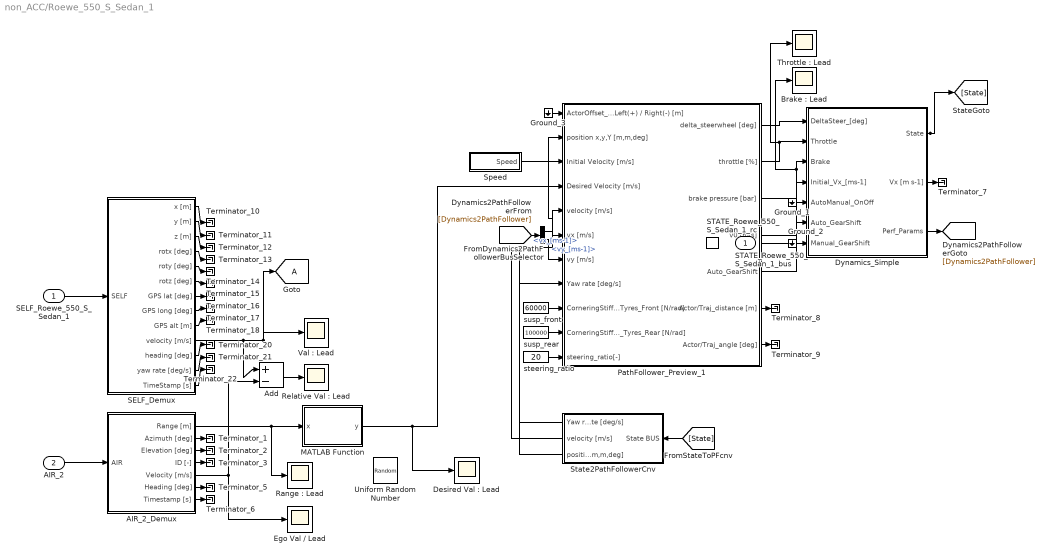
== system non_ACC/Roewe_550_S_Sedan_1 ==
  SELF_Roewe_550_S_Sedan_1 : Inport  Tag=inport/SelfPort  OutDataTypeStr=Bus: PRESCAN_SELFSENSORDATA  PortDimensions=1  SampleTime=1/20  BusOutputAsStruct=on
  AIR_2 : Inport  Tag=inport/AIR  Port=2  OutDataTypeStr=Bus: PRESCAN_AIRSENSORMESSAGE  PortDimensions=1  SampleTime=1/20  BusOutputAsStruct=on
  AIR_2_Demux : Subsystem  Tag=demux/AIR  mask(PreScan Demux Block: AIR){DetectionType=BBox, detectableObjects=1}
      mask prompts: DetectionType "Detection Type"; detectableObjects "Max. detectable objects"
      mask help:
      | The Actor Information Receiver sensor provides a fast, simple and generic detection solution which is not tied up to a specific technology and can be used for scenarios in which a simple sensor is needed.
      |
      | For more information, please click Help.
      mask init: same as non_ACC/Audi_A3_1/AIR_1_Demux
      settings: DeleteFcn=PreScanBlockDeleteFcn;
      mask Help: eval('openHelp(413)')
      mask TypeOptions DetectionType: Center | BBox | CoG
      mask Display:
      | disp(char('Det. type:         ',['{\it',DetectionTypeStr,'}']),'texmode','on')
      | port_label('output',1,'Range [m]')
      | port_label('output',2,'{\theta} [deg]','texmode','on')
      | port_label('output',3,'{\phi} [deg]','texmode','on')
      | port_label('output',4,'ID [-]','texmode','on')
      | port_label('output',5,'Velocity [m/s]','texmode','on')
      | port_label('output',6,'Heading [deg]','texmode','on')
      | port_label('output',7,'Timestamp [s]','texmode','on')
  Add : Sum  Inputs=+-
  "Brake : Lead" : Scope
  "Desired Val : Lead" : Scope
  Dynamics_Simple : Subsystem  Tag=Simple_Vehicle_Dynamics  mask(PreScan Block: Simple Dynamics){TimeStep=1/20, initialX=kea_demo_0218_cs_Roewe_550_S_Sedan_1_Dynamics_Simple_initialX, initialY=kea_demo_0218_cs_Roewe_550_S_Sedan_1_Dynamics_Simple_initialY, initialZ=kea_demo_0218_cs_Roewe_550_S_Sedan_1_Dynamics_Simple_initialZ, initialRoll=kea_demo_0218_cs_4669f259e7287783, initialPitch=kea_demo_0218_cs_87ee11d7829c0052, initialYaw=kea_demo_0218_cs_Roewe_550_S_Sedan_1_Dynamics_Simple_initialYaw}
      mask prompts: TimeStep "Auto assigned: Time Step [s]"; initialX "Ini x-position VEHICLE wrt GLOBAL axis system [m]"; initialY "Ini y-position VEHICLE wrt GLOBAL axis system [m]"; initialZ "Ini z-position VEHICLE wrt GLOBAL axis system [m]"; initialRoll "Ini roll-angle BODY wrt VEHICLE axis system [deg]"; initialPitch "Ini pitch-angle BODY wrt VEHICLE axis system [deg]"; initialYaw "Ini yaw-angle VEHICLE wrt GLOBAL axis system [deg]"
      mask help:
      | The Simple Dynamics Model is selected in the GUI to simulate vehicle dynamics behavior.
      |
      | The Simple Dynamics Model is completely open to the user. The parameters of this model can be set in the Simple Dynamics dialog in the GUI.
      |
      | For more information, please click Help.
      mask init:
      | p = SimpleDyn_pars;
      settings: DeleteFcn=PreScanBlockDeleteFcn;
      mask Help: eval('openHelp(220)')
      mask Display:
      | image(imread('SimpleDyn.png'))
      | port_label('input', 1, '{\delta}_S_t_ _e_e_r [deg]','texmode','on')
      | port_label('input', 2, 'Throttle [%]')
      | port_label('input', 3, 'Brake Pres [bar]')
      | port_label('input', 4, 'V_0 [ms-1]','texmode','on')
      | port_label('input', 5, 'Auto=[0]/Manual=[1]')
      | port_label('input', 6, 'Auto_GearShift')
      | port_label('input', 7, 'Manual_GearShift')
      | port_label('output', 1, 'State')
      | port_label('output', 2, 'Vx [ms-1]')
      | port_label('output', 3, 'Perf Params')
  Ego Val / Lead : Scope
  FromDynamics2PathFollowerBusSelector : BusSelector  OutputSignals=vx_[ms-1],vy_[ms-1]
  Ground_1 : Ground
  Ground_2 : Ground
  Ground_3 : Ground
  MATLAB Function : MATLAB Function  TreatAsAtomicUnit=on
  PathFollower_Preview_1 : Subsystem  Tag=PathFollower_Preview  LoadFcn=load PrescanXYZData;  mask(PreScan Block: Path Follower with Preview){LongCtrl_P=20, LongCtrl_I=0.3, LongCtrl_D=3.065, LongCtrl_AWU=1, LongCtrlDefault_P=20, LongCtrlDefault_I=0.3, LongCtrlDefault_D=3.065, LongCtrlDefault_AWU=1, PathUniqueID=kea_demo_0218_cs_1d5c9b61e8e009e5, mass=1532, Jzz=2700, length_a=1.115, length_l=2.705, Angle_Max_SteeringWheel=500, PreviewTime=1, DelayTime=0.1, LowSpeedLimit=20, MaxSteeringRate=1200, CSSampleTime=1/20, PFIntegrationFrequency=20}
      mask prompts: LongCtrl_P "Longitudinal Controller P"; LongCtrl_I "Longitudinal Controller I"; LongCtrl_D "Longitudinal Controller D"; LongCtrl_AWU "Longitudinal Controller AWU"; PathUniqueID "Path Unique ID"; mass "Mass vehicle total [kg]"; Jzz "Inertia vehicle around yaw axis [kg m2]"; length_a "Distance between COG and front axle [m]"; length_l "Length of wheelbase [m]"; Angle_Max_SteeringWheel "Maximum steering wheel angle [deg]"; PreviewTime "Preview time [s]"; DelayTime "Delay time [s]"; LowSpeedLimit "Low-speed limit [km/h]"; MaxSteeringRate "Maximum steering wheel angle rate [deg/s]"; CSSampleTime "Compilation Sheet sample time [s]"; PFIntegrationFrequency "Lateral controller frequency [Hz]"
      mask help:
      | The Path Follower Model is selected in the GUI to simulate driver behavior.
      |
      | For more information, please click Help.
      mask init:
      | RefreshCounter = max(floor((1/CSSampleTime) / (PFIntegrationFrequency)), 1);
      | PathFollowerBlockPath = gcb;
      mask Help: eval('openHelp(233)')
      mask DialogControl Container12 Prompt: Controller Parameters
      mask DialogControl Control2 Prompt: Reset PID parameters
      mask DialogControl Control2 Callback:
      | LongCtrlDefault_P = get_param(gcb,'LongCtrlDefault_P');
      | set_param(gcb,'LongCtrl_P',LongCtrlDefault_P);
      | 
      | LongCtrlDefault_I = get_param(gcb,'LongCtrlDefault_I');
      | set_param(gcb,'LongCtrl_I',LongCtrlDefault_I);
      | 
      | LongCtrlDefault_D = get_param(gcb,'LongCtrlDefault_D');
      | set_param(gcb,'LongCtrl_D',LongCtrlDefault_D);
      | 
      | LongCtrlDefault_AWU = get_param(gcb,'LongCtrlDefault_AWU');
      | set_param(gcb,'LongCtrl_AWU',LongCtrlDefault_AWU);
      mask DialogControl Container10 Prompt: System Parameters
  "Range : Lead" : Scope
  "Relative Val : Lead" : Scope
  SELF_Demux : Subsystem  Tag=demux/SelfPort  mask(PreScan Demux Block:){}
      mask help:
      | The SELF port shows (state) information of the actor itself. The outputs are position in the experiment's axis system and the GPS coordinates, and the object's absolute velocity and compass heading.
      |
      | For more information, please click Help.
      settings: DeleteFcn=PreScanBlockDeleteFcn;
      mask Help: eval('openHelp(462)')
      mask Display:
      | port_label('output',1,'x [m]')
      | port_label('output',2,'y [m]')
      | port_label('output',3,'z [m]','texmode','on')
      | port_label('output',4,'Rotx [deg]','texmode','on')
      | port_label('output',5,'Roty [deg]','texmode','on')
      | port_label('output',6,'Rotz [deg]','texmode','on')
      | port_label('output',7,'GPS lat [deg]','texmode','on')
      | port_label('output',8,'GPS long [deg]','texmode','on')
      | port_label('output',9,'GPS alt [m]','texmode','on')
      | port_label('output',10,'Velocity [m/s]')
      | port_label('output',11,'Heading [deg]')
      | port_label('output',12,'Yaw rate [deg/s]')
      | port_label('output',13,'Timestamp [s]')
  STATE_Roewe_550_S_Sedan_1_rc : RateTransition  Tag=mux_rc/StatePort  OutPortSampleTimeOpt=Inherit
  Speed : Subsystem
      settings: OpenFcn=open_system([gcb '/sfun'],'mask')
  State2PathFollowerCnv : Subsystem  Tag=State2PFConnection/cnv
  Terminator_{1..3,5..18,20..22} (20 alike) : Terminator
  "Throttle : Lead" : Scope
  Uniform Random Number : UniformRandomNumber  Minimum=13  Maximum=15  SampleTime=1
  "Val : Lead" : Scope
  steering_ratio : Constant  Tag=steering_ratio  Value=20
  susp_front : Constant  Tag=susp_front  Value=60000
  susp_rear : Constant  Tag=susp_rear  Value=100000
  STATE_Roewe_550_S_Sedan_1_bus : Outport  Tag=outport/StatePort  OutDataTypeStr=Bus: PRESCAN_STATEACTUATORDATA  PortDimensions=1  SampleTime=1/20
  tag scope: A=global
  wires:
  AIR_2_Demux/1(Range [m]) -> "Range : Lead"/1, MATLAB Function/1(x)
  MATLAB Function/1(y) -> "Desired Val : Lead"/1, PathFollower_Preview_1/4(Desired Velocity [m/s])
  STATE_Roewe_550_S_Sedan_1_rc/1 -> STATE_Roewe_550_S_Sedan_1_bus/1
  SELF_Roewe_550_S_Sedan_1/1 -> SELF_Demux/1(SELF)
  AIR_2/1 -> AIR_2_Demux/1(AIR)
  susp_front/1 -> PathFollower_Preview_1/9(CorneringStiffness_Tyres_Front [N/rad])
  susp_rear/1 -> PathFollower_Preview_1/10(CorneringStiffness_Tyres_Rear [N/rad])
  steering_ratio/1 -> PathFollower_Preview_1/11(steering_ratio[-])
  Speed/1(Speed) -> PathFollower_Preview_1/3(Initial Velocity [m/s])
  Dynamics_Simple/1(State) -> [State], STATE_Roewe_550_S_Sedan_1_rc/1
  [State] -> State2PathFollowerCnv/1(State BUS)
  State2PathFollowerCnv/1(Yaw rate [deg/s]) -> PathFollower_Preview_1/8(Yaw rate [deg/s])
  State2PathFollowerCnv/2(velocity [m/s]) -> PathFollower_Preview_1/5(velocity [m/s])
  State2PathFollowerCnv/3(position x,y,Y [m,m,deg]) -> PathFollower_Preview_1/2(position x,y,Y [m,m,deg])
  PathFollower_Preview_1/1(delta_steerwheel [deg]) -> Dynamics_Simple/1(DeltaSteer_[deg])
  PathFollower_Preview_1/2(throttle [%]) -> "Throttle : Lead"/1, Dynamics_Simple/2(Throttle)
  PathFollower_Preview_1/3(brake pressure [bar]) -> "Brake : Lead"/1, Dynamics_Simple/3(Brake)
  PathFollower_Preview_1/4(v0 [m/s]) -> Dynamics_Simple/4(Initial_Vx_[ms-1])
  PathFollower_Preview_1/5(Auto_GearShift) -> Dynamics_Simple/6(Auto_GearShift)
  Dynamics_Simple/3(Perf_Params) -> [Dynamics2PathFollower]
  FromDynamics2PathFollowerBusSelector/1 -> PathFollower_Preview_1/6(vx [m/s])  "<vx_[ms-1]>"
  FromDynamics2PathFollowerBusSelector/2 -> PathFollower_Preview_1/7(vy [m/s])  "<vy_[ms-1]>"
  [Dynamics2PathFollower] -> FromDynamics2PathFollowerBusSelector/1
  AIR_2_Demux/2(Azimuth [deg]) -> Terminator_1/1
  AIR_2_Demux/3(Elevation [deg]) -> Terminator_2/1
  AIR_2_Demux/4(ID [-]) -> Terminator_3/1
  AIR_2_Demux/6(Heading [deg]) -> Terminator_5/1
  AIR_2_Demux/7(Timestamp [s]) -> Terminator_6/1
  Ground_1/1 -> Dynamics_Simple/5(AutoManual_OnOff)
  Ground_2/1 -> Dynamics_Simple/7(Manual_GearShift)
  Dynamics_Simple/2(Vx [m s-1]) -> Terminator_7/1
  Ground_3/1 -> PathFollower_Preview_1/1(ActorOffset_Left(+) / Right(-) [m])
  PathFollower_Preview_1/6(Actor/Traj_distance [m]) -> Terminator_8/1
  PathFollower_Preview_1/7(Actor/Traj_angle [deg]) -> Terminator_9/1
  SELF_Demux/1(x [m]) -> Terminator_10/1
  SELF_Demux/2(y [m]) -> Terminator_11/1
  SELF_Demux/3(z [m]) -> Terminator_12/1
  SELF_Demux/4(rotx [deg]) -> Terminator_13/1
  SELF_Demux/5(roty [deg]) -> Terminator_14/1
  SELF_Demux/6(rotz [deg]) -> Terminator_15/1
  SELF_Demux/7(GPS lat [deg]) -> Terminator_16/1
  SELF_Demux/8(GPS long [deg]) -> Terminator_17/1
  SELF_Demux/9(GPS alt [m]) -> Terminator_18/1
  SELF_Demux/11(heading [deg]) -> Terminator_20/1
  SELF_Demux/12(yaw rate [deg/s]) -> Terminator_21/1
  SELF_Demux/13(TimeStamp [s]) -> Terminator_22/1
  AIR_2_Demux/5(Velocity [m/s]) -> Add/2, Ego Val / Lead/1
  Add/1 -> "Relative Val : Lead"/1
  SELF_Demux/10(velocity [m/s]) -> Add/1, [A], "Val : Lead"/1

== system non_ACC/SELF_Audi_A3_1 ==
  Sensor : S-Function  FunctionName=sfun_SelfSensor  Parameters=mbxruntime.parameters.convert(UniqueID), mbxruntime.parameters.convert(TimeStep)  SFunctionDeploymentMode=off  EnableBusSupport=off  mask(PreScan Source Block: SELF){UniqueID=189, TimeStep=1/20}
      mask prompts: UniqueID "Auto-Assigned: Unique ID"; TimeStep "Auto-Assigned: Upload Period [s]"
      mask help:
      | The SELF port shows (state) information of the actor itself. The outputs are position in the experiment's axis system and the GPS coordinates, and the object's absolute velocity and compass heading.
      |
      | For more information, please click Help.
      mask Help: eval('openHelp(462)')
      mask Display: image(imread('GPS.png'))
  SELF_Audi_A3_1 : Outport  Tag=outport/SelfPort  OutDataTypeStr=Bus: PRESCAN_SELFSENSORDATA  PortDimensions=1  SampleTime=1/20
  wires:
  Sensor/1 -> SELF_Audi_A3_1/1

== system non_ACC/SELF_Roewe_550_S_Sedan_1 ==
  Sensor : S-Function  FunctionName=sfun_SelfSensor  Parameters=mbxruntime.parameters.convert(UniqueID), mbxruntime.parameters.convert(TimeStep)  SFunctionDeploymentMode=off  EnableBusSupport=off  mask(PreScan Source Block: SELF){UniqueID=192, TimeStep=1/20}
      mask prompts: UniqueID "Auto-Assigned: Unique ID"; TimeStep "Auto-Assigned: Upload Period [s]"
      mask help:
      | The SELF port shows (state) information of the actor itself. The outputs are position in the experiment's axis system and the GPS coordinates, and the object's absolute velocity and compass heading.
      |
      | For more information, please click Help.
      mask Help: eval('openHelp(462)')
      mask Display: image(imread('GPS.png'))
  SELF_Roewe_550_S_Sedan_1 : Outport  Tag=outport/SelfPort  OutDataTypeStr=Bus: PRESCAN_SELFSENSORDATA  PortDimensions=1  SampleTime=1/20
  wires:
  Sensor/1 -> SELF_Roewe_550_S_Sedan_1/1

== system non_ACC/STATE_Audi_A3_1_bus ==
  STATE_Audi_A3_1_bus : Inport  Tag=inport/StatePort  OutDataTypeStr=Bus: PRESCAN_STATEACTUATORDATA  PortDimensions=1  SampleTime=1/20  BusOutputAsStruct=on
  Actuator : S-Function  FunctionName=sfun_StateActuator  Parameters=mbxruntime.parameters.convert(UniqueID), mbxruntime.parameters.convert(TimeStep)  SFunctionDeploymentMode=off  EnableBusSupport=off  mask(PreScan Sink Block: State){UniqueID=189, TimeStep=1/20}
      mask prompts: UniqueID "Auto-Assigned: Unique ID"; TimeStep "Auto-Assigned: Upload Period [s]"
      mask help:
      | The Actor State contains a vector signal of size (9x1), containing the following signals:
      |
      | -  Position    	(x,y,z)             	[m]
      | -  Velocity    	(vx,vy,vz)         	[m/s]
      | -  Angles       	(Roll, Pitch, Yaw)	[rad]
      |
      | The Actor state is defined in the global axis system.
      | The state is superponed on the Initial position defined in the GUI.
      |
      | For more information, please click Help.
      mask Help: eval('openHelp(222)')
      mask Display: image(imread('State.png'))
  wires:
  STATE_Audi_A3_1_bus/1 -> Actuator/1

== system non_ACC/STATE_Roewe_550_S_Sedan_1_bus ==
  STATE_Roewe_550_S_Sedan_1_bus : Inport  Tag=inport/StatePort  OutDataTypeStr=Bus: PRESCAN_STATEACTUATORDATA  PortDimensions=1  SampleTime=1/20  BusOutputAsStruct=on
  Actuator : S-Function  FunctionName=sfun_StateActuator  Parameters=mbxruntime.parameters.convert(UniqueID), mbxruntime.parameters.convert(TimeStep)  SFunctionDeploymentMode=off  EnableBusSupport=off  mask(PreScan Sink Block: State){UniqueID=192, TimeStep=1/20}
      mask prompts: UniqueID "Auto-Assigned: Unique ID"; TimeStep "Auto-Assigned: Upload Period [s]"
      mask help:
      | The Actor State contains a vector signal of size (9x1), containing the following signals:
      |
      | -  Position    	(x,y,z)             	[m]
      | -  Velocity    	(vx,vy,vz)         	[m/s]
      | -  Angles       	(Roll, Pitch, Yaw)	[rad]
      |
      | The Actor state is defined in the global axis system.
      | The state is superponed on the Initial position defined in the GUI.
      |
      | For more information, please click Help.
      mask Help: eval('openHelp(222)')
      mask Display: image(imread('State.png'))
  wires:
  STATE_Roewe_550_S_Sedan_1_bus/1 -> Actuator/1

== system non_ACC/ScenarioEngine ==
  Clock1 : Clock
  Stop Simulation : Stop
  sfun_ScenarioEngine1 : S-Function  FunctionName=sfun_ScenarioEngine  Parameters=TimeStep  SFunctionDeploymentMode=off  EnableBusSupport=off
  wires:
  sfun_ScenarioEngine1/1 -> Stop Simulation/1
  Clock1/1 -> sfun_ScenarioEngine1/1

== system non_ACC/Synchronizer ==
  Bus Selector1 : BusSelector  OutputSignals=FederateStopped
  Stop Simulation : Stop
  sfun_Synchronizer : S-Function  FunctionName=sfun_Synchronizer  Parameters=SampleTime  SFunctionDeploymentMode=off  EnableBusSupport=off  mask(Legacy Function){SFunctionSpec=void prescan_synchronizer_outputFcn(void ** work1, PRESCAN_SYNCHRONIZEDATA y1[1]), SampleTime=TimeStep, ShowSpec=on}
      mask prompts: SampleTime "Sample time (-1 for inherited):"; ShowSpec "Display function specification"
      mask help:
      | This block allows you to call the legacy functions specified by the following Legacy Code Tool definition:
      | def.SFunctionName = 'sfun_Synchronizer';
      | def.OutputFcnSpec = 'void prescan_synchronizer_outputFcn(void ** work1, PRESCAN_TIMESTAMPDATA u1[1], PRESCAN_SYNCHRONIZEDATA y1[1])';
      | def.StartFcnSpec = 'void prescan_synchronizer_startFcn(void ** work1)';
      | def.TerminateFcnSpec = 'void prescan_synchronizer_terminateFcn(void ** work1)';
      | def.HeaderFiles = {'prescan_synchronizer_data.h'};
      | def.HostLibFiles = {'sensorinterfaced.lib'};
      | def.IncPaths = {'src', 'C:\prescandev\vislibrary\vis\..\pimp\include\sensors\InterfaceRTW'};
      | def.SrcPaths = {'src'};
      | def.LibPaths = {'C:\\prescandev\\vislibrary_build\lib'};
      | def.SampleTime = 'parameterized';
      | def.Options.language = 'C';
      mask Help: <p>This block was generated automatically by the Legacy Code Tool. For detailed help on this tool, call<a href="matlab:legacy_code('help')"> legacy_code('help')</a>.</p>
      mask Callback ShowSpec:
      | if strcmp(get_param(gcbh, 'ShowSpec'), 'on')
      |   set_param(gcbh, 'MaskDisplay', sprintf('fprintf(''%s'');', get_param(gcbh, 'SFunctionSpec')));
      | else
      |   set_param(gcbh, 'MaskDisplay', sprintf('fprintf(''%s'');', get_param(gcbh, 'FunctionName')));
      | end
      mask Display: fprintf('void prescan_synchronizer_outputFcn(void ** work1, PRESCAN_SYNCHRONIZEDATA y1[1])');
  wires:
  sfun_Synchronizer/1 -> Bus Selector1/1
  Bus Selector1/1 -> Stop Simulation/1  "<FederateStopped>"

== system non_ACC/Audi_A3_1/ACC System ==
  Distance : Inport
  Ego val : Inport  Port=2
  Gain : Gain  Gain=1.6
  If : If  IfExpression=u1==1  ElseIfExpressions=u1==2, u1==3
  If Action Subsystem : Subsystem  TreatAsAtomicUnit=on
  If Action Subsystem1 : Subsystem  TreatAsAtomicUnit=on
  If Action Subsystem2 : Subsystem  TreatAsAtomicUnit=on
  If Action Subsystem3 : Subsystem  TreatAsAtomicUnit=on
  MATLAB Function : MATLAB Function  TreatAsAtomicUnit=on
  Merge : Merge  Inputs=4
  Merge1 : Merge  Inputs=4
  throttle : Outport
  brake : Outport  Port=2
  wires:
  Ego val/1 -> MATLAB Function/2(u2), If Action Subsystem2/1(Ego val), If Action Subsystem1/1(Ego val), If Action Subsystem3/1(Ego val)
  If/1 -> If Action Subsystem/Action
  If/4 -> If Action Subsystem1/Action
  If Action Subsystem1/1(throttle) -> Merge/4
  If Action Subsystem/2(brake) -> Merge1/1
  If Action Subsystem1/2(brake) -> Merge1/4
  MATLAB Function/1(y) -> If/1
  Distance/1 -> Gain/1
  Gain/1 -> MATLAB Function/1(u1)
  If/2 -> If Action Subsystem2/Action
  If Action Subsystem2/1(throttle) -> Merge/2
  If Action Subsystem2/2(brake) -> Merge1/2
  If/3 -> If Action Subsystem3/Action
  If Action Subsystem3/1(throttle) -> Merge/3
  If Action Subsystem3/2(brake) -> Merge1/3
  Merge1/1 -> brake/1
  Merge/1 -> throttle/1
  If Action Subsystem/1(throttle) -> Merge/1
